simulink model "Simulink"  (R2025a)
settings: Solver=ode4  StartTime=0.0  StopTime=10  FixedStep=P.Ts_plant  RelTol=1e-3
values from neighbouring files (symbols this model uses):
  P = block.DialogPrm(1).Data;block.NumDworks=1    [ctrl.m]    (also in hydro_core.m = varargin{2}; varargout{1}=s(7); obs.m = block.DialogPrm(1).Data;hydro_core('validate',P); para.m = struct; plant.m = block.DialogPrm(1).Data)
settings Model: Creator=leejx  LastModifiedBy=leejx

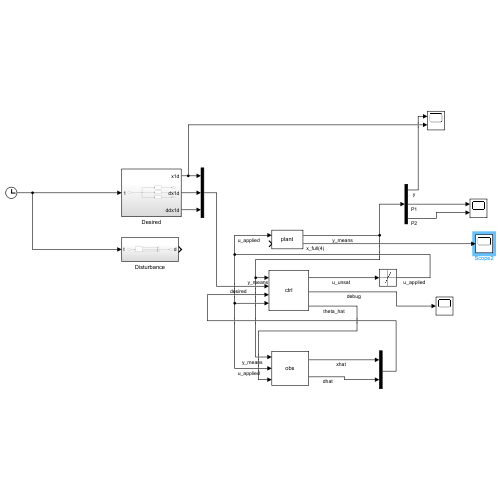
[thumbnail: Simulink's stored preview of the top-level diagram]
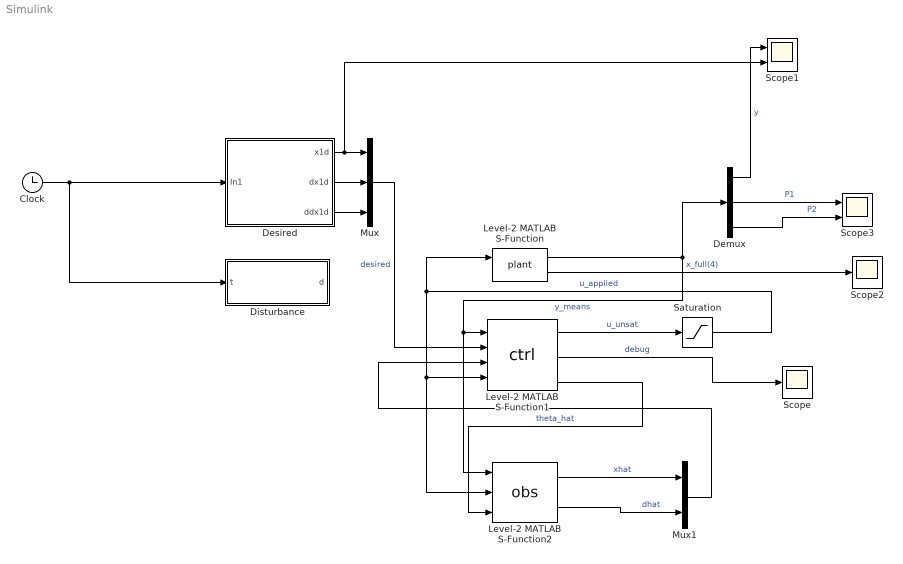
== system Simulink ==
  Clock : Clock
  Demux : Demux  Outputs=3
  Desired : Subsystem
  Disturbance : Subsystem
  Level-2 MATLAB S-Function : M-S-Function  FunctionName=plant  Parameters=P
  Level-2 MATLAB S-Function1 : M-S-Function  FunctionName=ctrl  Parameters=P
  Level-2 MATLAB S-Function2 : M-S-Function  FunctionName=obs  Parameters=P
  Mux : Mux  Inputs=3
  Mux1 : Mux  Inputs=2
  Saturation : Saturate  UpperLimit=P.u_max  LowerLimit=-P.u_max
  Scope : Scope
  Scope1 : Scope  NumInputPorts=2
      settings: ActiveDisplayYMinimum=-0.083670498363984547  ActiveDisplayYMaximum=0.25448203860324281
  Scope2 : Scope
      settings: ActiveDisplayYMinimum=-7.14354859890084E+6  ActiveDisplayYMaximum=1.4131634398838423E+7  DataLoggingVariableName=ScopeData2
  Scope3 : Scope  NumInputPorts=2
      settings: ActiveDisplayYMinimum=2.023738443972744E+6  ActiveDisplayYMaximum=8.1709977497858908E+6  DataLoggingVariableName=ScopeData3
  wires:
  Clock/1 -> Disturbance/1(t), Desired/1(In1)
  Level-2 MATLAB S-Function1/1 -> Saturation/1  "u_unsat"
  Level-2 MATLAB S-Function1/3 -> Level-2 MATLAB S-Function2/3  "theta_hat"
  Level-2 MATLAB S-Function1/2 -> Scope/1  "debug"
  Level-2 MATLAB S-Function2/1 -> Mux1/1  "xhat"
  Level-2 MATLAB S-Function2/2 -> Mux1/2  "dhat"
  Saturation/1 -> Level-2 MATLAB S-Function1/4, Level-2 MATLAB S-Function2/2, Level-2 MATLAB S-Function/1  "u_applied"
  Mux/1 -> Level-2 MATLAB S-Function1/2  "desired"
  Desired/2(dx1d) -> Mux/2
  Desired/1(x1d) -> Scope1/2, Mux/1
  Desired/3(ddx1d) -> Mux/3
  Mux1/1 -> Level-2 MATLAB S-Function1/3
  Level-2 MATLAB S-Function/1 -> Demux/1, Level-2 MATLAB S-Function2/1, Level-2 MATLAB S-Function1/1  "y_means"
  Level-2 MATLAB S-Function/2 -> Scope2/1  "x_full(4)"
  Demux/1 -> Scope1/1  "y"
  Demux/2 -> Scope3/1  "P1"
  Demux/3 -> Scope3/2  "P2"

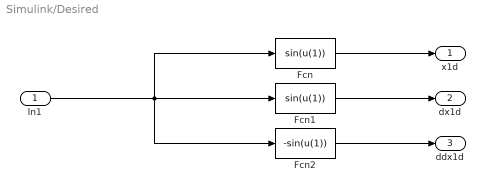
== system Simulink/Desired ==
  In1 : Inport
  Fcn : Fcn  Expr=sin(u(1))
  Fcn1 : Fcn  Expr=sin(u(1))
  Fcn2 : Fcn  Expr=-sin(u(1))
  x1d : Outport
  dx1d : Outport  Port=2
  ddx1d : Outport  Port=3
  wires:
  Fcn/1 -> x1d/1
  Fcn1/1 -> dx1d/1
  In1/1 -> Fcn2/1, Fcn1/1, Fcn/1
  Fcn2/1 -> ddx1d/1

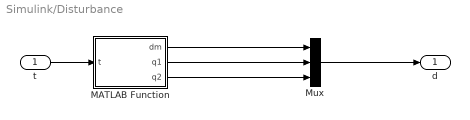
== system Simulink/Disturbance ==
  t : Inport
  MATLAB Function : MATLAB Function  TreatAsAtomicUnit=on
  Mux : Mux  Inputs=3
  d : Outport
  wires:
  t/1 -> MATLAB Function/1(t)
  Mux/1 -> d/1
  MATLAB Function/1(dm) -> Mux/1
  MATLAB Function/2(q1) -> Mux/2
  MATLAB Function/3(q2) -> Mux/3

== matlab function Simulink/Disturbance/MATLAB Function ==
  data: t input; dm output; q1 output; q2 output
function [dm,q1,q2] = dist_wave(t)
% 输入：t，仿真时间，单位 s
% 输出：三个实际扰动信号
% 以下幅值为初步仿真设置，不是设备辨识结果。

% 扰动力：1 s后平滑加入，幅值100 N，频率0.7 Hz
t_force = max(t - 1, 0);
b_force = 1 - exp(-(t_force / 0.2)^4);
dm = 100 * b_force * sin(2*pi*0.7*t_force);

% 流量扰动：2 s后平滑加入，幅值1e-7 m^3/s，频率0.3 Hz
t_flow = max(t - 2, 0);
b_flow = 1 - exp(-(t_flow / 0.2)^4);
q1 = 1e-7 * b_flow * sin(2*pi*0.3*t_flow);

% 初步采用两腔相等的等效流量扰动
q2 = q1;
end
